simulink model "roll_model_TRUCKSIM_18DOF_REVISED"  (R2023b)
settings: Solver=FixedStepAuto  StartTime=0.0  StopTime=20  FixedStep=0.0005  RelTol=1e-3
StopFcn:
  | save_dataset_18state;
libraries: Solver_SF x1
(part 1 of 5)
settings Model: Creator=duong  LastModifiedBy=ThinkPad
settings SolverCC: AlgebraicLoopSolver=TrustRegion
settings DataIOCC: ReturnWorkspaceOutputs=off
settings SFSimCC: CustomCodeUndefinedFunction=UseInterfaceOnly

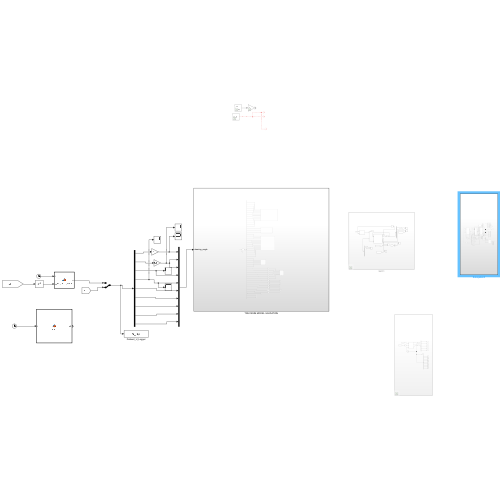
[thumbnail: Simulink's stored preview of the top-level diagram]
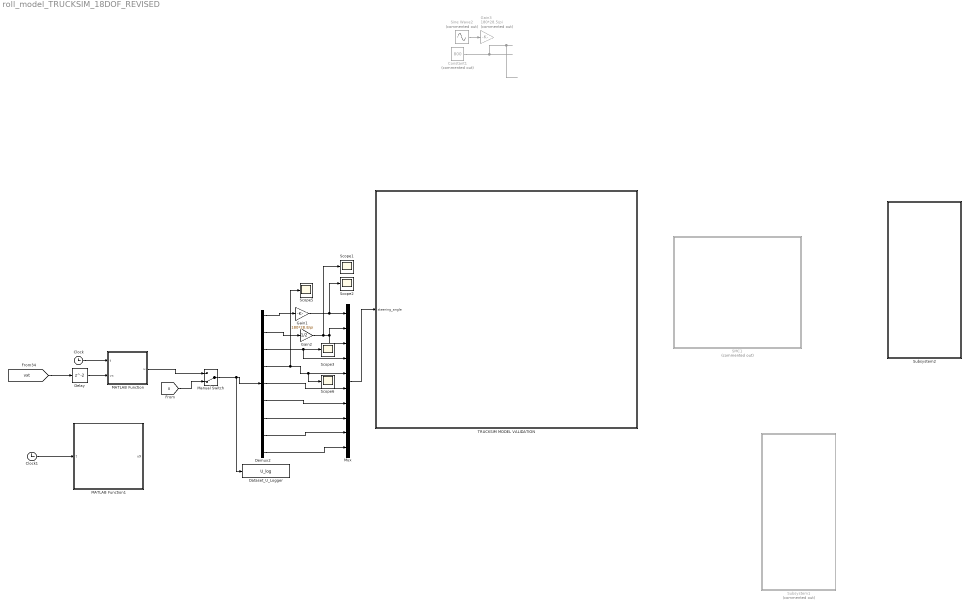
== system roll_model_TRUCKSIM_18DOF_REVISED ==
  Clock : Clock
      settings: Decimation=20
  Clock1 : Clock
      settings: Decimation=20
  Constant1 : Constant  Commented=on  Value=800
  Dataset_U_Logger : ToWorkspace  VariableName=U_log  SampleTime=-1
  Delay : Delay
  Demux2 : Demux  Outputs=9
  Gain1 : Gain  Gain=180*28.8/pi
  Gain2 : Gain  Gain=1/2
  Gain3 : Gain  Commented=on  Gain=180*28.5/pi
  MATLAB Function : MATLAB Function  TreatAsAtomicUnit=on
  MATLAB Function1 : MATLAB Function  TreatAsAtomicUnit=on
  Manual Switch : ManualSwitch  CurrentSetting=0
  Mux : Mux  Inputs=10
  SMC1 : Subsystem  Commented=on
  Scope{1..3,5..6} (5 alike) : Scope
  Sine Wave2 : Sin  Commented=on  Amplitude=0.01  SampleTime=0
  Subsystem1 : Subsystem  Commented=on
  Subsystem2 : Subsystem
  TRUCKSIM MODEL VALIDATION : Subsystem
  wires:
  Mux/1 -> TRUCKSIM MODEL VALIDATION/1(steering_angle)
  Constant1/1 -> ?
  Sine Wave2/1 -> Gain3/1
  Gain2/1 -> Scope1/1, Mux/3, Mux/2
  Demux2/2 -> Gain2/1
  Gain1/1 -> Scope2/1, Mux/1
  Demux2/4 -> Scope5/1, Scope6/1, Mux/5
  Demux2/5 -> Mux/6
  Demux2/6 -> Mux/7
  Demux2/7 -> Mux/8
  Demux2/8 -> Mux/9
  Demux2/9 -> Mux/10
  Clock/1 -> MATLAB Function/1(t)
  [vxt] -> Delay/1
  Delay/1 -> MATLAB Function/2(vx)
  Manual Switch/1 -> Demux2/1, Dataset_U_Logger/1
  [u] -> Manual Switch/2
  Clock1/1 -> MATLAB Function1/1(t)
  Demux2/1 -> Gain1/1
  MATLAB Function/1(u) -> Manual Switch/1
  Demux2/3 -> Mux/4, Scope3/1

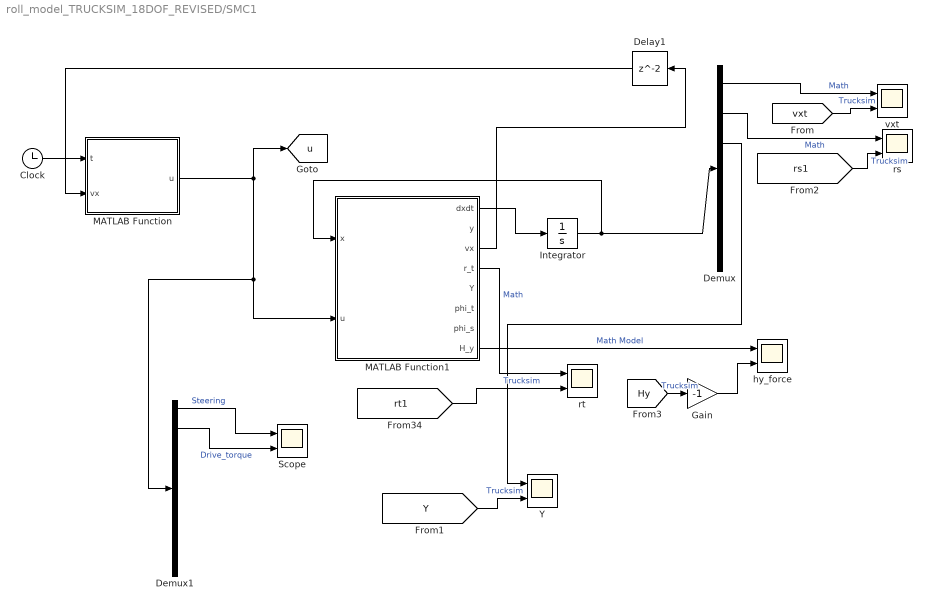
== system roll_model_TRUCKSIM_18DOF_REVISED/SMC1 ==
  Clock : Clock
      settings: Decimation=20
  Delay1 : Delay
  Demux : Demux  Outputs=18
  Demux1 : Demux  Outputs=9
  Gain : Gain  Gain=-1
  Integrator : Integrator  InitialCondition=[12;zeros(7,1);(12/0.51)*ones(6,1);zeros(4,1)]
  MATLAB Function : MATLAB Function  TreatAsAtomicUnit=on
  MATLAB Function1 : MATLAB Function  TreatAsAtomicUnit=on
  Scope : Scope  NumInputPorts=2
  Y : Scope  NumInputPorts=2
  hy_force : Scope  NumInputPorts=2
  rs : Scope  NumInputPorts=2
  rt : Scope  NumInputPorts=2
  vxt : Scope  NumInputPorts=2
  tag scope: u=global
  wires:
  Demux/7 -> Y/1
  MATLAB Function/1(u) -> MATLAB Function1/2(u), Demux1/1, [u]
  Demux1/1 -> Scope/1  "Steering"
  Demux1/2 -> Scope/2  "Drive_torque"
  [rs1] -> rs/2  "Trucksim"
  Demux/4 -> rs/1  "Math"
  [rt1] -> rt/2  "Trucksim"
  [Y] -> Y/2  "Trucksim"
  MATLAB Function1/3(vx) -> Delay1/1
  Delay1/1 -> MATLAB Function/2(vx)
  Demux/1 -> vxt/1  "Math"
  [vxt] -> vxt/2  "Trucksim"
  MATLAB Function1/4(r_t) -> rt/1  "Math"
  Clock/1 -> MATLAB Function/1(t)
  Integrator/1 -> MATLAB Function1/1(x), Demux/1
  MATLAB Function1/1(dxdt) -> Integrator/1
  MATLAB Function1/8(H_y) -> hy_force/1  "Math Model"
  [Hy] -> Gain/1  "Trucksim"
  Gain/1 -> hy_force/2

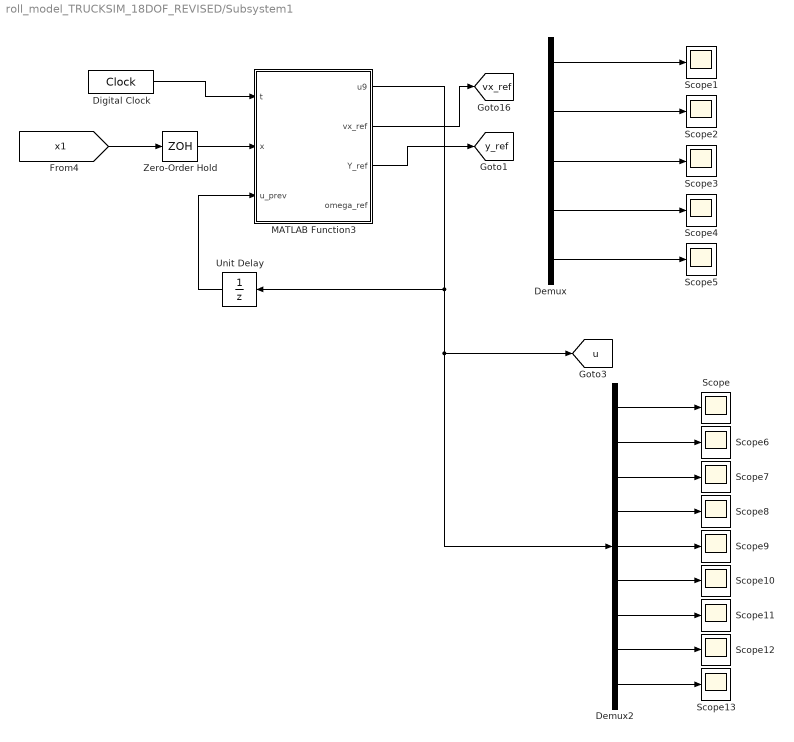
== system roll_model_TRUCKSIM_18DOF_REVISED/Subsystem1 ==
  Demux : Demux  Outputs=5
  Demux2 : Demux  Outputs=9
  Digital Clock : DigitalClock  SampleTime=0.01
  MATLAB Function3 : MATLAB Function  TreatAsAtomicUnit=on
  Scope{,1..13} (14 alike) : Scope
  Unit Delay : UnitDelay  InitialCondition=zeros(9,1)  SampleTime=0.01  HasFrameUpgradeWarning=on
  Zero-Order Hold : ZeroOrderHold  SampleTime=0.01
  tag scope: u=global, vx_ref=global, y_ref=global
  wires:
  Demux2/9 -> Scope13/1
  Demux2/8 -> Scope12/1
  Demux2/7 -> Scope11/1
  Demux2/6 -> Scope10/1
  Demux2/5 -> Scope9/1
  Demux2/4 -> Scope8/1
  Demux2/3 -> Scope7/1
  Demux2/2 -> Scope6/1
  Demux2/1 -> Scope/1
  Demux/5 -> Scope5/1
  Demux/4 -> Scope4/1
  Demux/3 -> Scope3/1
  Demux/2 -> Scope2/1
  Demux/1 -> Scope1/1
  MATLAB Function3/1(u9) -> Unit Delay/1, Demux2/1, [u]
  [x1] -> Zero-Order Hold/1
  Zero-Order Hold/1 -> MATLAB Function3/2(x)
  Unit Delay/1 -> MATLAB Function3/3(u_prev)
  Digital Clock/1 -> MATLAB Function3/1(t)
  MATLAB Function3/2(vx_ref) -> [vx_ref]
  MATLAB Function3/3(Y_ref) -> [y_ref]

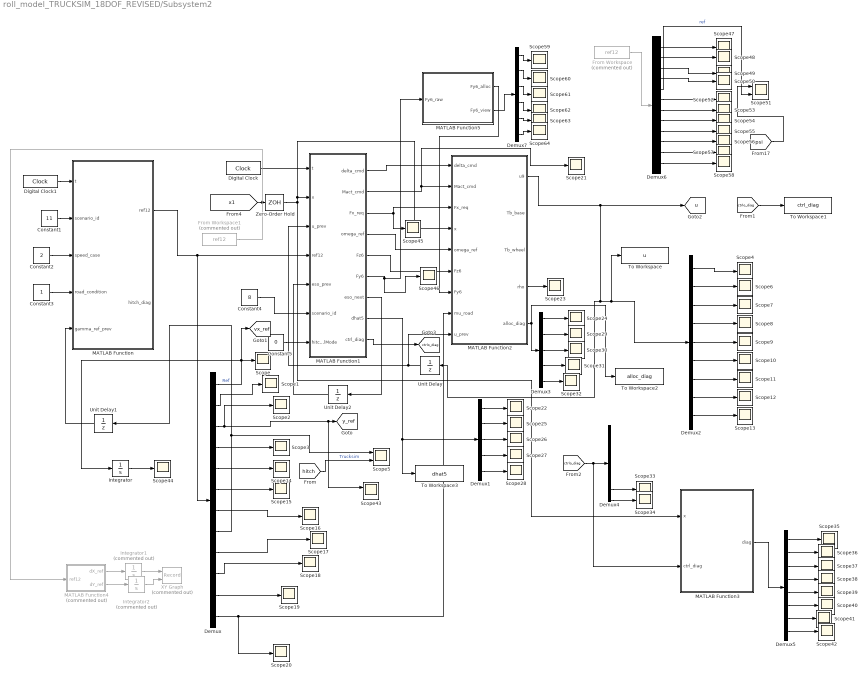
== system roll_model_TRUCKSIM_18DOF_REVISED/Subsystem2 ==
  Constant1 : Constant  Value=11
  Constant2 : Constant  Value=2
  Constant3 : Constant
  Constant4 : Constant  Value=8
  Constant5 : Constant  Value=0
  Demux : Demux  Outputs=12
  Demux1 : Demux  Outputs=5
  Demux2 : Demux  Outputs=9
  Demux3 : Demux  Outputs=5
  Demux4 : Demux  Outputs=8
  Demux5 : Demux  Outputs=8
  Demux6 : Demux  Outputs=12
  Demux7 : Demux  Outputs=6
  Digital Clock : DigitalClock  SampleTime=0.01
  Digital Clock1 : DigitalClock  SampleTime=0.01
  From Workspace : FromWorkspace  Commented=on  VariableName=ref12
  From Workspace1 : FromWorkspace  Commented=on  VariableName=ref12
  Integrator : Integrator
  Integrator1 : Integrator  Commented=on
  Integrator2 : Integrator  Commented=on
  MATLAB Function : MATLAB Function  TreatAsAtomicUnit=on
  MATLAB Function1 : MATLAB Function  TreatAsAtomicUnit=on
  MATLAB Function2 : MATLAB Function  TreatAsAtomicUnit=on
  MATLAB Function3 : MATLAB Function  TreatAsAtomicUnit=on
  MATLAB Function4 : MATLAB Function  Commented=on  TreatAsAtomicUnit=on
  MATLAB Function5 : MATLAB Function  TreatAsAtomicUnit=on
  Scope{,1..4,6..42,44..50,52..64} (62 alike) : Scope
  Scope43 : Scope  NumInputPorts=2
  Scope5 : Scope  NumInputPorts=2
  Scope51 : Scope  NumInputPorts=2
  To Workspace : ToWorkspace  VariableName=u  SaveFormat=Timeseries  SampleTime=-1
  To Workspace1 : ToWorkspace  VariableName=ctrl_diag  SaveFormat=Timeseries  SampleTime=-1
  To Workspace2 : ToWorkspace  VariableName=alloc_diag  SaveFormat=Timeseries  SampleTime=-1
  To Workspace3 : ToWorkspace  VariableName=dhat5  SaveFormat=Timeseries  SampleTime=-1
  Unit Delay : UnitDelay  InitialCondition=zeros(9,1)  SampleTime=0.01  HasFrameUpgradeWarning=on
  Unit Delay1 : UnitDelay  SampleTime=0.01  HasFrameUpgradeWarning=on
  Unit Delay2 : UnitDelay  InitialCondition=zeros(10,1)  SampleTime=0.01  HasFrameUpgradeWarning=on
  XY Graph : Record  Commented=on  FileSettingsInternal="{\"entries\":[{\"content\":{\"excelSettings\":{\"content\":{},\"type\":\"Streamout.ExcelSettings\"}},\"type\":\"Streamout.FileSettingStorage\",\"uuid\":\"\"}],\"packageUris\":[\"http:\\/\\/schema.mathworks.com\\/mf0\\/streamout_blocks\\/R2020a\"],\"version\":\"1.0\"}"  Layout=[1 1]  SignalsInternal="{\"entries\":[{\"content\":{},\"type\":\"RecordBlkView.InputSignals\",\"uuid\":\"\"}],\"packageUris\":[\"http:\\/\\/schema.mathworks.com\\/mf0\\/streamout_blocks\\/R2020a\"],\"version\":\"1.0\"}"  VisualizationBindings="{\"xyplotplugin\":{\"info\":[{\"series\":[],\"subplotID\":1}]}}"  CompatibilityTag=XY
  Zero-Order Hold : ZeroOrderHold  SampleTime=0.01
  tag scope: ctrlo_diag=global, u=global, vx_ref=global, y_ref=global
  wires:
  Digital Clock/1 -> MATLAB Function1/1(t)
  Zero-Order Hold/1 -> MATLAB Function1/2(x), MATLAB Function2/4(x), MATLAB Function3/1(x)
  [x1] -> Zero-Order Hold/1
  Digital Clock1/1 -> MATLAB Function/1(t)
  Constant1/1 -> MATLAB Function/2(scenario_id)
  Constant2/1 -> MATLAB Function/3(speed_case)
  Constant3/1 -> MATLAB Function/4(road_condition)
  MATLAB Function1/1(delta_cmd) -> MATLAB Function2/1(delta_cmd)
  MATLAB Function1/2(Mact_cmd) -> Scope21/1, MATLAB Function2/2(Mact_cmd)
  MATLAB Function1/3(Fx_req) -> Scope45/1, MATLAB Function2/3(Fx_req)
  MATLAB Function1/4(omega_ref) -> MATLAB Function2/5(omega_ref)
  MATLAB Function1/5(Fz6) -> MATLAB Function2/6(Fz6)
  MATLAB Function1/6(Fy6) -> MATLAB Function5/1(Fy6_raw), Scope46/1
  MATLAB Function2/1(u9) -> Unit Delay/1, To Workspace/1, Demux2/1, [u]
  Demux/1 -> [vx_ref], Integrator/1, Scope/1
  Demux/2 -> Scope1/1
  Demux/3 -> Scope2/1, Scope43/1, [y_ref]
  Demux/4 -> Scope3/1
  Unit Delay/1 -> MATLAB Function1/3(u_prev), MATLAB Function2/9(u_prev)
  Demux2/5 -> Scope9/1
  Demux2/2 -> Scope6/1
  Demux2/3 -> Scope7/1
  Demux2/7 -> Scope11/1
  Demux2/1 -> Scope4/1
  Demux2/8 -> Scope12/1
  Demux2/4 -> Scope8/1
  Demux2/6 -> Scope10/1
  Demux2/9 -> Scope13/1
  Demux/8 -> Scope5/1, Unit Delay1/1  "Ref"
  Unit Delay1/1 -> MATLAB Function/5(gamma_ref_prev)
  MATLAB Function1/7(eso_next) -> Unit Delay2/1
  Unit Delay2/1 -> MATLAB Function1/5(eso_prev)
  [hitch] -> Scope5/2  "Trucksim"
  Demux/5 -> Scope14/1
  Demux/6 -> Scope15/1
  Demux/7 -> Scope16/1
  Demux/9 -> Scope17/1
  Demux/10 -> Scope18/1
  Demux/11 -> Scope19/1
  Demux/12 -> MATLAB Function2/8(mu_road), Scope20/1
  MATLAB Function1/8(dhat5) -> To Workspace3/1, Demux1/1
  MATLAB Function2/4(rho) -> Scope23/1
  MATLAB Function2/5(alloc_diag) -> Demux3/1, To Workspace2/1
  Demux1/1 -> Scope22/1
  Demux1/2 -> Scope25/1
  Demux1/3 -> Scope26/1
  Demux1/4 -> Scope27/1
  Demux1/5 -> Scope28/1
  Demux3/1 -> Scope24/1
  Demux3/2 -> Scope29/1
  Demux3/3 -> Scope30/1
  Demux3/4 -> Scope31/1
  Demux3/5 -> Scope32/1
  [ctrlo_diag] -> MATLAB Function3/2(ctrl_diag), Demux4/1
  Demux4/7 -> Scope33/1
  Demux4/8 -> Scope34/1
  MATLAB Function3/1(diag) -> Demux5/1
  Demux5/1 -> Scope35/1
  Demux5/2 -> Scope36/1
  Demux5/3 -> Scope37/1
  Demux5/4 -> Scope38/1
  Demux5/5 -> Scope39/1
  Demux5/6 -> Scope40/1
  Demux5/7 -> Scope41/1
  Demux5/8 -> Scope42/1
  [ctrlo_diag] -> To Workspace1/1
  Integrator/1 -> Scope44/1
  MATLAB Function4/1(dX_ref) -> Integrator1/1
  MATLAB Function4/2(dY_ref) -> Integrator2/1
  Integrator1/1 -> XY Graph/1
  Integrator2/1 -> XY Graph/2
  MATLAB Function1/9(ctrl_diag) -> [ctrlo_diag]
  Constant4/1 -> MATLAB Function1/6(scenario_id)
  From Workspace/1 -> Demux6/1
  Demux6/1 -> Scope47/1
  Demux6/2 -> Scope48/1
  Demux6/3 -> Scope49/1
  Demux6/4 -> Scope50/1
  Demux6/5 -> Scope51/2  "ref"
  Demux6/6 -> Scope52/1
  Demux6/7 -> Scope53/1
  Demux6/8 -> Scope54/1
  Demux6/9 -> Scope55/1
  Demux6/10 -> Scope56/1
  Demux6/11 -> Scope57/1
  Demux6/12 -> Scope58/1
  From Workspace1/1 -> MATLAB Function4/1(ref12)
  [psi] -> Scope51/1
  Constant5/1 -> MATLAB Function1/7(hitchControlMode)
  MATLAB Function5/2(Fy6_view) -> Demux7/1
  Demux7/1 -> Scope59/1
  Demux7/2 -> Scope60/1
  Demux7/3 -> Scope61/1
  Demux7/4 -> Scope62/1
  Demux7/5 -> Scope63/1
  Demux7/6 -> Scope64/1
  MATLAB Function5/1(Fy6_alloc) -> MATLAB Function2/7(Fy6)
  MATLAB Function/1(ref12) -> MATLAB Function1/4(ref12), Demux/1

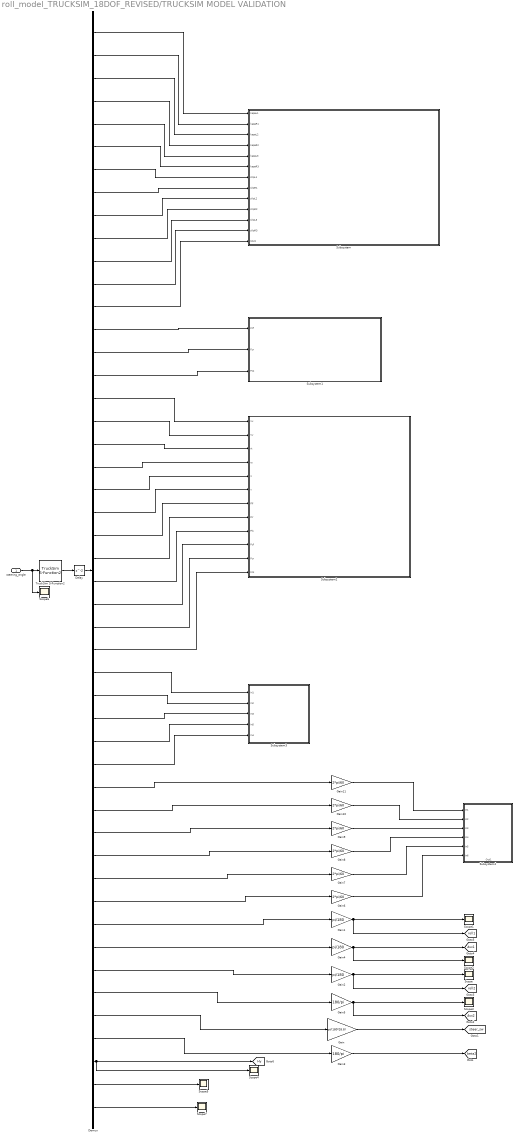
== system roll_model_TRUCKSIM_18DOF_REVISED/TRUCKSIM MODEL VALIDATION ==
  steering_angle : Inport
  Delay : Delay
  Demux : Demux  Outputs=48
  Gain : Gain  Gain=pi/(180*28.8)
  Gain1 : Gain  Gain=pi/180
  Gain{6..11} (6 alike) : Gain  Gain=2*pi/60
  Gain2 : Gain  Gain=pi/180
  Gain3 : Gain  Gain=180/pi
  Gain4 : Gain  Gain=pi/180
  Gain5 : Gain  Gain=180/pi
  Scope{,1..7} (8 alike) : Scope
  Subsystem : Subsystem
  Subsystem1 : Subsystem
  Subsystem2 : Subsystem
  Subsystem3 : Subsystem
  Subsystem4 : Subsystem
      settings: PortSchema="{\"entries\":[{\"content\":{\"sides\":[{\"content\":{\"connectorIds\":[\"In1\",\"In2\",\"In3\",\"In4\",\"In5\",\"In6\"]},\"type\":\"ConnectorPlacement.EquallySpacedRectSide\",\"uuid\":\"070411b8-1eaf-4600-ae67-312ecabb46ce\"},{\"content\":{\"side\":\"RIGHT\"},\"type\":\"ConnectorPlacement.EquallySpacedRectSide\",\"uuid\":\"e64aaffe-29d9-425a-a5f7-83ef24fd6d70\"},{\"content\":{\"side\":\"TOP\"},\"type\":\"ConnectorPlacement.EquallySpacedRectSide\",\"uuid\":\"b5ab375b-6b47-4d88-bc86-a6bac8bdcf5b\"},{\"content\":{\"connectorIds\":[\"Out1\"],\"side\":\"BOTTOM\"},\"type\":\"ConnectorPlacement.EquallySpacedRectSide\",\"uuid\":\"71cf385b-1b44-4da4-ba17-2e03fc073379\"}]},\"type\":\"ConnectorPlacement.EquallySpacedConnector\",\"uuid\":\"3bbbd5e1-cd10-4b5e-b773-54af9b41425b\"}],\"packageUris\":[\"http://schema.mathworks.com/mf0/Connector/R2020b\"],\"version\":\"1.0\"}"
  TruckSim S-Function2 : Solver_SF/TruckSim S-Function2  Priority=1  VehicleCode=s_s  SIMFILE=simfile.sim
      settings: AttributesFormatString=Vehicle Code: %<VehicleCode>  SourceProductName=TruckSim S-Function
  tag scope: Avx1=global, Avx2=global, Hy=global, beta2=global, roll1=global, roll2=global, steer_sw=global
  wires:
  steering_angle/1 -> TruckSim S-Function2/1, Scope6/1
  Demux/19 -> Subsystem2/3(rt)
  Demux/13 -> Subsystem/13(hitch)
  Demux/6 -> Subsystem/6(kapaR3)
  Delay/1 -> Demux/1
  Gain3/1 -> [beta2]
  Demux/35 -> Gain10/1
  Demux/12 -> Subsystem/12(slipR3)
  TruckSim S-Function2/1 -> Delay/1
  Gain11/1 -> Subsystem4/1(In1)
  Demux/40 -> Gain1/1
  Demux/5 -> Subsystem/5(kapaL3)
  Gain10/1 -> Subsystem4/2(In2)
  Demux/18 -> Subsystem2/2(Vy)
  Demux/4 -> Subsystem/4(kapaR2)
  Demux/46 -> Scope4/1, [Hy]
  Demux/29 -> Subsystem3/1(In1)
  Demux/1 -> Subsystem/1(kapaL1)
  Demux/3 -> Subsystem/3(kapaL2)
  Demux/2 -> Subsystem/2(kapaR1)
  Demux/7 -> Subsystem/7(slipL1)
  Gain/1 -> [steer_sw]
  Demux/21 -> Subsystem2/5(X)
  Demux/17 -> Subsystem2/1(Vx)
  Demux/8 -> Subsystem/8(slipR1)
  Demux/9 -> Subsystem/9(slipL2)
  Demux/10 -> Subsystem/10(slipR2)
  Gain7/1 -> Subsystem4/5(In5)
  Demux/39 -> Gain6/1
  Demux/11 -> Subsystem/11(slipL3)
  Demux/44 -> Gain/1
  Demux/36 -> Gain9/1
  Demux/27 -> Subsystem2/11(Fcr)
  Demux/14 -> Subsystem1/1(Fzf)
  Gain4/1 -> [Avx1], Scope2/1
  Gain1/1 -> [roll1], Scope1/1
  Demux/43 -> Gain5/1
  Demux/15 -> Subsystem1/2(Fzr)
  Gain9/1 -> Subsystem4/3(In3)
  Demux/32 -> Subsystem3/4(In5)
  Demux/16 -> Subsystem1/3(Fzs)
  Demux/42 -> Gain2/1
  Demux/26 -> Subsystem2/10(Fcf)
  Demux/20 -> Subsystem2/4(rs)
  Gain6/1 -> Subsystem4/6(In6)
  Demux/38 -> Gain7/1
  Demux/28 -> Subsystem2/12(Fcs)
  Demux/22 -> Subsystem2/6(Y)
  Demux/30 -> Subsystem3/2(In2)
  Demux/23 -> Subsystem2/7(Flf)
  Demux/41 -> Gain4/1
  Demux/24 -> Subsystem2/8(Flr)
  Gain8/1 -> Subsystem4/4(In4)
  Demux/45 -> Gain3/1
  Demux/25 -> Subsystem2/9(Fls)
  Demux/37 -> Gain8/1
  Demux/33 -> Subsystem3/5(In4)
  Demux/31 -> Subsystem3/3(In3)
  Demux/34 -> Gain11/1
  Gain5/1 -> Scope3/1, [Avx2]
  Gain2/1 -> Scope/1, [roll2]
  Demux/47 -> Scope5/1
  Demux/48 -> Scope7/1

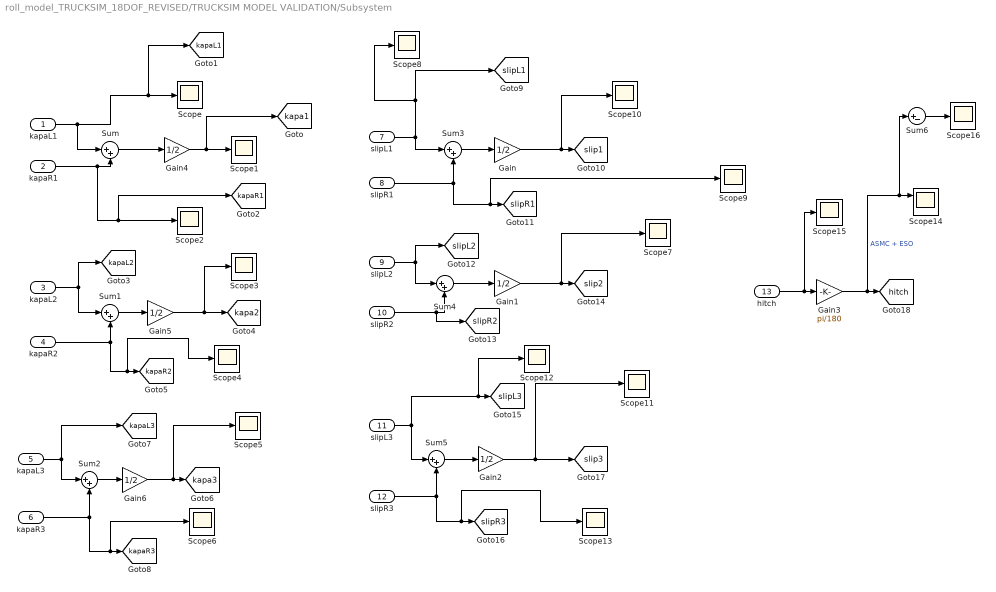
== system roll_model_TRUCKSIM_18DOF_REVISED/TRUCKSIM MODEL VALIDATION/Subsystem ==
  kapaL1 : Inport
  kapaR1 : Inport  Port=2
  kapaL2 : Inport  Port=3
  kapaR2 : Inport  Port=4
  kapaL3 : Inport  Port=5
  kapaR3 : Inport  Port=6
  slipL1 : Inport  Port=7
  slipR1 : Inport  Port=8
  slipL2 : Inport  Port=9
  slipR2 : Inport  Port=10
  slipL3 : Inport  Port=11
  slipR3 : Inport  Port=12
  hitch : Inport  Port=13
  Gain{,1..2,4..6} (6 alike) : Gain  Gain=1/2
  Gain3 : Gain  Gain=pi/180
  Scope{,1..13,15..16} (16 alike) : Scope
  Scope14 : Scope  NumInputPorts=2
  Sum{,1..5} (6 alike) : Sum  Inputs=|++
  Sum6 : Sum  Inputs=|+-
  tag scope: hitch=global, kapa1=global, kapa2=global, kapa3=global, kapaL1=global, kapaL2=global, kapaL3=global, kapaR1=global, kapaR2=global, kapaR3=global, slip1=global, slip2=global, slip3=global, slipL1=global, slipL2=global, slipL3=global, slipR1=global, slipR2=global, slipR3=global
  wires:
  kapaL1/1 -> Scope/1, [kapaL1], Sum/1
  kapaR1/1 -> [kapaR1], Scope2/1, Sum/2
  Sum/1 -> Gain4/1
  kapaL2/1 -> [kapaL2], Sum1/1
  kapaR2/1 -> Scope4/1, [kapaR2], Sum1/2
  Sum1/1 -> Gain5/1
  kapaL3/1 -> [kapaL3], Sum2/1
  kapaR3/1 -> Scope6/1, [kapaR3], Sum2/2
  Sum2/1 -> Gain6/1
  slipL1/1 -> Scope8/1, [slipL1], Sum3/1
  slipR1/1 -> Scope9/1, [slipR1], Sum3/2
  Sum3/1 -> Gain/1
  Gain/1 -> Scope10/1, [slip1]
  slipL2/1 -> [slipL2], Sum4/1
  slipR2/1 -> [slipR2], Sum4/2
  Sum4/1 -> Gain1/1
  Gain1/1 -> Scope7/1, [slip2]
  slipL3/1 -> Scope12/1, [slipL3], Sum5/1
  slipR3/1 -> Scope13/1, [slipR3], Sum5/2
  Sum5/1 -> Gain2/1
  Gain2/1 -> Scope11/1, [slip3]
  hitch/1 -> Scope15/1, Gain3/1
  Gain3/1 -> Sum6/1, Scope14/1, [hitch]  "ASMC + ESO"
  Gain4/1 -> [kapa1], Scope1/1
  Gain5/1 -> [kapa2], Scope3/1
  Gain6/1 -> Scope5/1, [kapa3]
  Sum6/1 -> Scope16/1

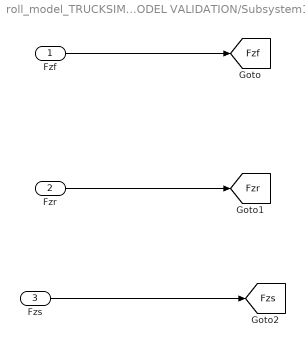
== system roll_model_TRUCKSIM_18DOF_REVISED/TRUCKSIM MODEL VALIDATION/Subsystem1 ==
  Fzf : Inport
  Fzr : Inport  Port=2
  Fzs : Inport  Port=3
  tag scope: Fzf=global, Fzr=global, Fzs=global
  wires:
  Fzf/1 -> [Fzf]
  Fzr/1 -> [Fzr]
  Fzs/1 -> [Fzs]

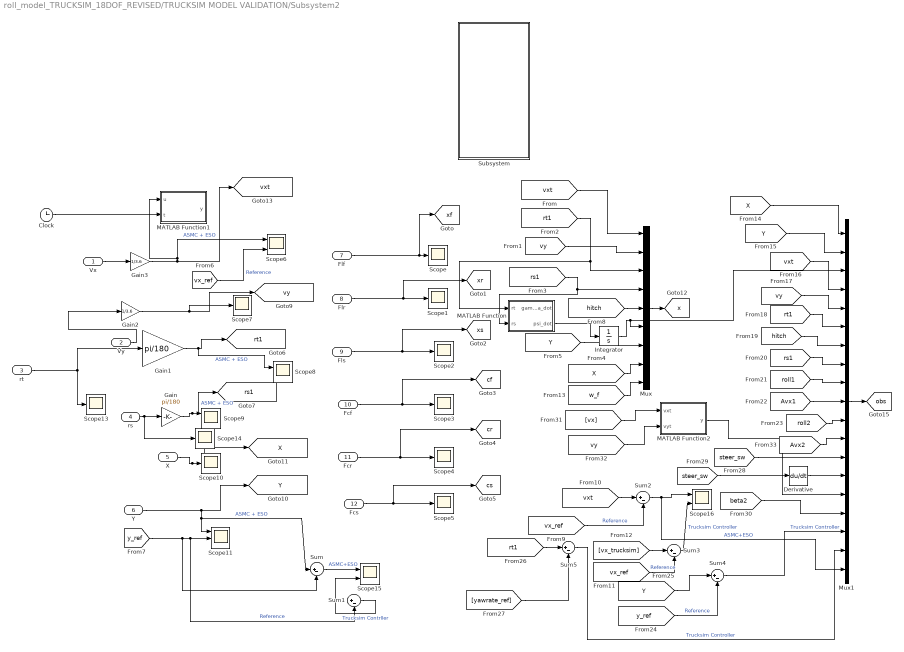
== system roll_model_TRUCKSIM_18DOF_REVISED/TRUCKSIM MODEL VALIDATION/Subsystem2 ==
  Vx : Inport
  Vy : Inport  Port=2
  rt : Inport  Port=3
  rs : Inport  Port=4
  X : Inport  Port=5
  Y : Inport  Port=6
  Flf : Inport  Port=7
  Flr : Inport  Port=8
  Fls : Inport  Port=9
  Fcf : Inport  Port=10
  Fcr : Inport  Port=11
  Fcs : Inport  Port=12
  Clock : Clock
      settings: Decimation=15
  Derivative : Derivative
  Gain : Gain  Gain=pi/180
  Gain1 : Gain  Gain=pi/180
  Gain2 : Gain  Gain=1/3.6
  Gain3 : Gain  Gain=1/3.6
  Integrator : Integrator
  MATLAB Function : MATLAB Function  TreatAsAtomicUnit=on
  MATLAB Function1 : MATLAB Function  TreatAsAtomicUnit=on
  MATLAB Function2 : MATLAB Function  TreatAsAtomicUnit=on
  Mux : Mux  Inputs=9
  Mux1 : Mux  Inputs=19
  Scope{,1..5,7,10,13..14} (10 alike) : Scope
  Scope11 : Scope  NumInputPorts=3
  Scope{6,8..9,15..16} (5 alike) : Scope  NumInputPorts=2
  Subsystem : Subsystem
  Sum{,1..5} (6 alike) : Sum  Inputs=|+-
  tag scope: X=global, Y=global, cf=global, cr=global, cs=global, obs=global, rs1=global, rt1=global, vxt=global, vy=global, x=global, xf=global, xr=global, xs=global
  wires:
  Fcf/1 -> [cf], Scope3/1
  Fcr/1 -> [cr], Scope4/1
  Fcs/1 -> [cs], Scope5/1
  Vx/1 -> Gain3/1
  Vy/1 -> Gain2/1
  rt/1 -> Scope13/1, Gain1/1
  rs/1 -> Scope14/1, Gain/1
  X/1 -> [X], Scope10/1
  Y/1 -> [Y], Scope11/1, Sum/1  "ASMC + ESO"
  Gain/1 -> [rs1], Scope9/1  "ASMC + ESO"
  Gain1/1 -> Scope8/1, [rt1]  "ASMC + ESO"
  Flr/1 -> [xr], Scope1/1
  Flf/1 -> [xf], Scope/1
  Fls/1 -> [xs], Scope2/1
  Gain2/1 -> [vy], Scope7/1
  Gain3/1 -> Scope6/1, MATLAB Function1/1(u), [vxt]  "ASMC + ESO"
  Clock/1 -> MATLAB Function1/2(t)
  [vxt] -> Mux/1
  [vy] -> Mux/2
  [rt1] -> Mux/3, MATLAB Function/1(rt)
  [rs1] -> Mux/4, MATLAB Function/2(rs)
  [X] -> Mux/8
  [Y] -> Mux/7
  Mux/1 -> [x]
  [y_ref] -> Sum/2, Sum1/2, Scope11/2  "Reference"
  [hitch] -> Mux/5
  Integrator/1 -> Mux1/3, Mux/6
  MATLAB Function/2(psi_dot) -> Integrator/1
  Sum/1 -> Scope15/1  "ASMC+ESO"
  Sum1/1 -> Scope15/2  "Trucksim Contrller"
  [vx_ref] -> Sum2/2  "Reference"
  [vxt] -> Sum2/1
  [vx_ref] -> Sum3/2  "Reference"
  [vx_trucksim] -> Sum3/1
  Sum2/1 -> Mux1/19, Scope16/1  "ASMC+ESO"
  Sum3/1 -> Scope16/2  "Trucksim Controller"
  [w_f] -> Mux/9
  [X] -> Mux1/1
  [Y] -> Mux1/2
  [vxt] -> Mux1/4
  [vy] -> Mux1/5
  [rt1] -> Mux1/6
  Mux1/1 -> [obs]
  [Y] -> Sum4/1
  [y_ref] -> Sum4/2  "Reference"
  Sum4/1 -> Mux1/17  "Trucksim Controller"
  [rt1] -> Sum5/1
  [yawrate_ref] -> Sum5/2
  Sum5/1 -> Mux1/18  "Trucksim Controller"
  [hitch] -> Mux1/7
  [rs1] -> Mux1/8
  [roll1] -> Mux1/9
  [Avx1] -> Mux1/10
  [roll2] -> Mux1/11
  [steer_sw] -> Derivative/1
  [beta2] -> Mux1/16
  [vx] -> MATLAB Function2/1(vxt)
  [vy] -> MATLAB Function2/2(vyt)
  MATLAB Function2/1(y) -> Mux1/15
  Derivative/1 -> Mux1/14
  [steer_sw] -> Mux1/13
  [Avx2] -> Mux1/12
  [vx_ref] -> Scope6/2  "Reference"

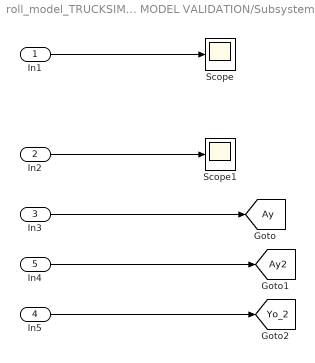
== system roll_model_TRUCKSIM_18DOF_REVISED/TRUCKSIM MODEL VALIDATION/Subsystem3 ==
  In1 : Inport
  In2 : Inport  Port=2
  In3 : Inport  Port=3
  In5 : Inport  Port=4
  In4 : Inport  Port=5
  Scope : Scope
  Scope1 : Scope
  tag scope: Ay2=global, Ay=global, Yo_2=global
  wires:
  In2/1 -> Scope1/1
  In1/1 -> Scope/1
  In3/1 -> [Ay]
  In4/1 -> [Ay2]
  In5/1 -> [Yo_2]

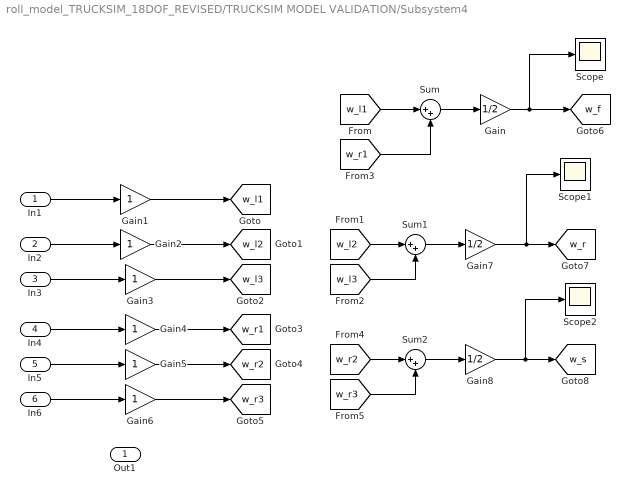
== system roll_model_TRUCKSIM_18DOF_REVISED/TRUCKSIM MODEL VALIDATION/Subsystem4 ==
  In1 : Inport
  In2 : Inport  Port=2
  In3 : Inport  Port=3
  In4 : Inport  Port=4
  In5 : Inport  Port=5
  In6 : Inport  Port=6
  Gain : Gain  Gain=1/2
  Gain{1..6} (6 alike) : Gain
  Gain7 : Gain  Gain=1/2
  Gain8 : Gain  Gain=1/2
  Scope : Scope
  Scope1 : Scope
  Scope2 : Scope
  Sum : Sum  Inputs=|++
  Sum1 : Sum  Inputs=|++
  Sum2 : Sum  Inputs=|++
  Out1 : Outport
  tag scope: w_f=global, w_l1=global, w_l2=global, w_l3=global, w_r1=global, w_r2=global, w_r3=global, w_r=global, w_s=global
  wires:
  [w_l1] -> Sum/1
  [w_r1] -> Sum/2
  Sum/1 -> Gain/1
  In1/1 -> Gain1/1
  Gain1/1 -> [w_l1]
  In2/1 -> Gain2/1
  Gain2/1 -> [w_l2]
  In3/1 -> Gain3/1
  Gain3/1 -> [w_l3]
  In4/1 -> Gain4/1
  Gain4/1 -> [w_r1]
  In5/1 -> Gain5/1
  Gain5/1 -> [w_r2]
  In6/1 -> Gain6/1
  Gain6/1 -> [w_r3]
  Gain/1 -> Scope/1, [w_f]
  Gain7/1 -> Scope1/1, [w_r]
  [w_l2] -> Sum1/1
  Sum1/1 -> Gain7/1
  [w_l3] -> Sum1/2
  Gain8/1 -> Scope2/1, [w_s]
  [w_r2] -> Sum2/1
  Sum2/1 -> Gain8/1
  [w_r3] -> Sum2/2

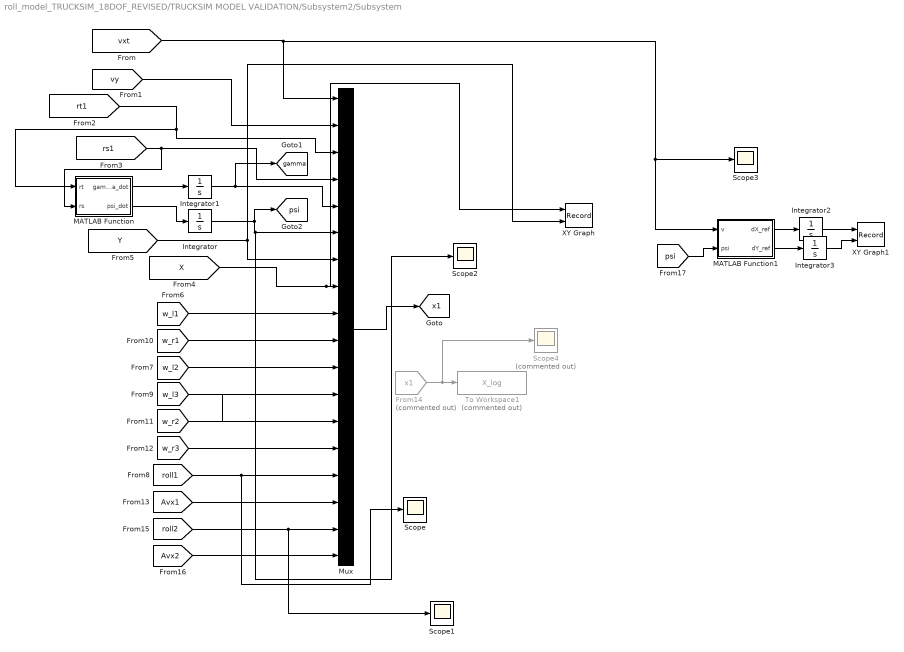
== system roll_model_TRUCKSIM_18DOF_REVISED/TRUCKSIM MODEL VALIDATION/Subsystem2/Subsystem ==
  From14 : From  Commented=on  GotoTag=x1  TagVisibility=global
  Integrator{,1..3} (4 alike) : Integrator
  MATLAB Function : MATLAB Function  TreatAsAtomicUnit=on
  MATLAB Function1 : MATLAB Function  TreatAsAtomicUnit=on
  Mux : Mux  Inputs=18
  Scope{,1..3} (4 alike) : Scope
  Scope4 : Scope  Commented=on
  To Workspace1 : ToWorkspace  Commented=on  VariableName=X_log  SampleTime=-1
  XY Graph : Record  FileSettingsInternal="{\"entries\":[{\"content\":{\"excelSettings\":{\"content\":{},\"type\":\"Streamout.ExcelSettings\"}},\"type\":\"Streamout.FileSettingStorage\",\"uuid\":\"\"}],\"packageUris\":[\"http:\\/\\/schema.mathworks.com\\/mf0\\/streamout_blocks\\/R2020a\"],\"version\":\"1.0\"}"  Layout=[1 1]  SignalsInternal="{\"entries\":[{\"content\":{\"signals\":[{\"content\":{\"blockPath\":[],\"dimensions\":[1],\"domain\":\"\",\"lineColor\":\"#a2142f\",\"plots\":[1],\"port\":1,\"sid\":[\"\"],\"signalID\":8528,\"signalName\":\"From4\"},\"type\":\"RecordBlkView.Signal\",\"uuid\":\"\"},{\"content\":{\"blockPath\":[],\"dimensions\":[1],\"domain\":\"\",\"lineColor\":\"#139fff\",\"plots\":[1],\"port\":2,\"sid\":[\"\"],\"signalID\":8532,\"signalName\":\"From5\"},\"type\":\"RecordBlkView.Signal\",\"uuid\":\"\"}]},\"type\":\"RecordBlkView.InputSignals\",\"uuid\":\"\"}],\"packageUris\":[\"http:\\/\\/schema.mathworks.com\\/mf0\\/streamout_blocks\\/R2020a\"],\"version\":\"1.0\"}"  VisualizationBindings="{\"xyplotplugin\":{\"info\":[{\"series\":[{\"bindingParametersList\":[{\"parameter\":\"X-Axis\",\"signalID\":8528,\"signalName\":\"From4\"},{\"parameter\":\"Y-Axis\",\"signalID\":8532,\"signalName\":\"From5\"}],\"seriesID\":4705}],\"subplotID\":1}]}}"  CompatibilityTag=XY
  XY Graph1 : Record  FileSettingsInternal="{\"entries\":[{\"content\":{\"excelSettings\":{\"content\":{},\"type\":\"Streamout.ExcelSettings\"}},\"type\":\"Streamout.FileSettingStorage\",\"uuid\":\"\"}],\"packageUris\":[\"http:\\/\\/schema.mathworks.com\\/mf0\\/streamout_blocks\\/R2020a\"],\"version\":\"1.0\"}"  Layout=[1 1]  SignalsInternal="{\"entries\":[{\"content\":{\"signals\":[{\"content\":{\"blockPath\":[],\"dimensions\":[1],\"domain\":\"\",\"lineColor\":\"#a2142f\",\"plots\":[1],\"port\":1,\"sid\":[\"\"],\"signalID\":8536,\"signalName\":\"Integrator2\"},\"type\":\"RecordBlkView.Signal\",\"uuid\":\"\"},{\"content\":{\"blockPath\":[],\"dimensions\":[1],\"domain\":\"\",\"lineColor\":\"#139fff\",\"plots\":[1],\"port\":2,\"sid\":[\"\"],\"signalID\":8540,\"signalName\":\"Integrator3\"},\"type\":\"RecordBlkView.Signal\",\"uuid\":\"\"}]},\"type\":\"RecordBlkView.InputSignals\",\"uuid\":\"\"}],\"packageUris\":[\"http:\\/\\/schema.mathworks.com\\/mf0\\/streamout_blocks\\/R2020a\"],\"version\":\"1.0\"}"  VisualizationBindings="{\"xyplotplugin\":{\"info\":[{\"series\":[{\"bindingParametersList\":[{\"parameter\":\"X-Axis\",\"signalID\":8536,\"signalName\":\"Integrator2\"},{\"parameter\":\"Y-Axis\",\"signalID\":8540,\"signalName\":\"Integrator3\"}],\"seriesID\":29226}],\"subplotID\":1}]}}"  CompatibilityTag=XY
  tag scope: gamma=global, psi=global, x1=global
  wires:
  MATLAB Function/2(psi_dot) -> Integrator/1
  [vy] -> Mux/2
  [X] -> XY Graph/1, Mux/8
  Integrator/1 -> [psi], Scope2/1, Mux/6
  [Y] -> XY Graph/2, Mux/7
  [rs1] -> MATLAB Function/2(rs), Mux/4
  [vxt] -> MATLAB Function1/1(v), Scope3/1, Mux/1
  [rt1] -> MATLAB Function/1(rt), Mux/3
  MATLAB Function/1(gamma_dot) -> Integrator1/1
  Integrator1/1 -> [gamma], Mux/5
  [w_l1] -> Mux/9
  [w_r1] -> Mux/10
  [w_l2] -> Mux/11
  [w_r3] -> Mux/14
  [roll1] -> Scope/1, Mux/15
  [Avx1] -> Mux/16
  Mux/1 -> [x1]
  From14/1 -> Scope4/1, To Workspace1/1
  [w_r2] -> Mux/12
  [w_l3] -> Mux/13
  [roll2] -> Scope1/1, Mux/17
  [Avx2] -> Mux/18
  [psi] -> MATLAB Function1/2(psi)
  MATLAB Function1/1(dX_ref) -> Integrator2/1
  Integrator2/1 -> XY Graph1/1
  MATLAB Function1/2(dY_ref) -> Integrator3/1
  Integrator3/1 -> XY Graph1/2

== matlab function roll_model_TRUCKSIM_18DOF_REVISED/Subsystem2/MATLAB Function3 ==
  data: x input; diag output; ctrl_diag input
function diag = fcn(x,ctrl_diag)
%#codegen

phi_t  = x(15);
dphi_t = x(16);

phi_s  = x(17);
dphi_s = x(18);

sPhiT = dphi_t + 3.0*phi_t;
sPhiS = dphi_s + 2.0*phi_s;

sRoll_calc = sPhiT + 0.30*sPhiS;

diag = zeros(8,1);

diag(1) = phi_t;
diag(2) = dphi_t;
diag(3) = phi_s;
diag(4) = dphi_s;

diag(5) = sPhiT;
diag(6) = sPhiS;
diag(7) = sRoll_calc;
diag(8) = sRoll_calc - ctrl_diag(7);
end

== matlab function roll_model_TRUCKSIM_18DOF_REVISED/Subsystem1/MATLAB Function3 ==
  data: t input; u9 output; x input; u_prev input; vx_ref output; Y_ref output; omega_ref output
function [u9,vx_ref,Y_ref,omega_ref] = fcn(t,x,u_prev)
%#codegen
% =========================================================================
% MODEL-ASSISTED SMC FOR FULL 18-STATE TRACTOR-SEMITRAILER
%
% FULL MODEL:
%   vehicle_18dof_full_roll(x,u)
%
% STATES:
% x(1)  = vx
% x(2)  = vy
% x(3)  = rt
% x(4)  = rs
% x(5)  = gamma
% x(6)  = psi
% x(7)  = Y
% x(8)  = X
%
% x(9)  = omega_fL
% x(10) = omega_fR
% x(11) = omega_rL
% x(12) = omega_rR
% x(13) = omega_sL
% x(14) = omega_sR
%
% x(15:18) = roll states
%
% PHYSICAL INPUT:
% u9(1) = delta
% u9(2) = Tdrive
% u9(3) = Mact
% u9(4) = Tb_fL
% u9(5) = Tb_fR
% u9(6) = Tb_rL
% u9(7) = Tb_rR
% u9(8) = Tb_sL
% u9(9) = Tb_sR
% =========================================================================


%% ========================================================================
% FIXED OUTPUT DIMENSIONS
% ========================================================================

u9 = zeros(9,1);

omega_ref = zeros(6,1);


%% ========================================================================
% CONTROLLER SAMPLE TIME
% ========================================================================

Ts = 0.01;


%% ========================================================================
% STATES
% ========================================================================

vx = x(1);

vy = x(2);

rt = x(3);

rs = x(4);

gamma = x(5);

psi = x(6);

Y = x(7);


omega_fL = x(9);
omega_fR = x(10);

omega_rL = x(11);
omega_rR = x(12);

omega_sL = x(13);
omega_sR = x(14);

% Roll states
phi_t  = x(15);
dphi_t = x(16);
phi_s  = x(17);
dphi_s = x(18);


%% ========================================================================
% REFERENCE GENERATOR
% ========================================================================

[vx_ref,ax_ref,Y_ref,dY_ref,psi_ref,rt_ref] = ...
    reference_local(t);


%% Reference one step ahead

[~,~,~,~,~,rt_ref_next] = ...
    reference_local(t+Ts);


dr_ref = ...
    (rt_ref_next-rt_ref)/Ts;


%% ========================================================================
% FULL 18-STATE MODEL
%
% This is the important difference from the previous simple SMC.
%
% The controller now explicitly uses the nonlinear plant model.
% ========================================================================

[xdot_model,y_model] = ...
    vehicle_18dof_full_roll(x,u_prev);


%% Model-predicted accelerations

ax_model = ...
    xdot_model(1);


dr_model = ...
    xdot_model(3);


Ydot_model = ...
    xdot_model(7);

% Model-predicted roll accelerations
ddphi_t_model = xdot_model(16);
ddphi_s_model = xdot_model(18);

% Model-predicted load-transfer ratios
LTR_f_model = y_model(6);
LTR_r_model = y_model(7);
LTR_s_model = y_model(47); %#ok<NASGU>

if abs(LTR_f_model) >= abs(LTR_r_model)
    LTR_t_model = LTR_f_model;
else
    LTR_t_model = LTR_r_model;
end


%% ========================================================================
% VEHICLE PARAMETERS
% ========================================================================

m_t = 5760.0;

m_s = 6640.0;

m = ...
    m_t+m_s;


%% Geometry

Lf = 1.305130208;

Lr = 2.194869792;

L = ...
    Lf+Lr;


Tf = 2.030;

Tr = 1.863;

Ts_track = 1.863;


%% Wheel radii

Rf = 0.51;

Rr = 0.51;

Rs = 0.51;


%% ========================================================================
% 1. MODEL-ASSISTED LONGITUDINAL SMC
% ========================================================================

ev = ...
    vx-vx_ref;


%% Desired longitudinal acceleration

kv = ...
    29.2;


Kv = ...
    2.75;


phi_v = ...
    0.6;


ax_des = ...
      ax_ref ...
    - kv*ev ...
    - Kv*satfun(ev/phi_v);


%% ------------------------------------------------------------------------
% Convert previous physical actuators to approximate total Fx
% -------------------------------------------------------------------------

Fx_prev = ...
    u_prev(2)/Rf;


Fx_prev = ...
    Fx_prev ...
    - u_prev(4)/Rf ...
    - u_prev(5)/Rf ...
    - u_prev(6)/Rr ...
    - u_prev(7)/Rr ...
    - u_prev(8)/Rs ...
    - u_prev(9)/Rs;


%% ------------------------------------------------------------------------
% Model-assisted correction
%
% Delta Fx = m * (desired acceleration - model acceleration)
% -------------------------------------------------------------------------

dFx = ...
    m*(ax_des-ax_model);


Fx_target = ...
    Fx_prev+dFx;


%% Force limits

if Fx_target > 15000.0

    Fx_target = 15000.0;

elseif Fx_target < -15000.0

    Fx_target = -15000.0;

end


%% ========================================================================
% 2. MODEL-ASSISTED LATERAL SMC
% ========================================================================

eY = ...
    Y-Y_ref;


eYdot = ...
    Ydot_model-dY_ref;


epsi = ...
    wrap_pi(psi-psi_ref);


er = ...
    rt-rt_ref;


%% Sliding surface

lambda_Y = ...
    0.90;


lambda_Ydot = ...
    0.82;


lambda_psi = ...
    1.00;


s_lat = ...
      er ...
    + lambda_psi*epsi ...
    + lambda_Y*eY ...
    + lambda_Ydot*eYdot;


%% ========================================================================
% DESIRED YAW ACCELERATION
% ========================================================================

Kr = ...
    2.5;


Kpsi = ...
    1.2;


KY = ...
    0.4;


KYdot = ...
    0.35;


Ksw = ...
    0.7;


phi_lat = ...
    0.2;


dr_des = ...
      dr_ref ...
    - Kr*er ...
    - Kpsi*epsi ...
    - KY*eY ...
    - KYdot*eYdot ...
    - Ksw*satfun(s_lat/phi_lat);


%% ========================================================================
% STEERING SENSITIVITY FROM FULL NONLINEAR MODEL
%
% Numerically estimate:
%
%       d(dr_t)/d(delta)
%
% using vehicle_18dof_full_roll itself.
% ========================================================================

delta_previous = ...
    u_prev(1);


delta_probe = ...
    0.20*pi/180.0;


u_probe = ...
    u_prev;


delta_probe_value = ...
    delta_previous+delta_probe;


delta_max = ...
    5.0*pi/180.0;


if delta_probe_value > delta_max

    delta_probe_value = delta_max;

end


u_probe(1) = ...
    delta_probe_value;


xdot_probe = ...
    vehicle_18dof_full_roll(x,u_probe);


dr_probe = ...
    xdot_probe(3);


d_delta = ...
    delta_probe_value-delta_previous;


if abs(d_delta) > 1.0e-8

    Bdelta = ...
        (dr_probe-dr_model)/d_delta;

else

    Bdelta = ...
        0.0;

end


%% ========================================================================
% MODEL-INVERSE STEERING
% ========================================================================

if abs(Bdelta) > 0.20

    delta_model = ...
        delta_previous ...
        +(dr_des-dr_model)/Bdelta;

else

    delta_model = ...
        delta_previous;

end


%% Limit model inversion

if delta_model > delta_max

    delta_model = delta_max;

elseif delta_model < -delta_max

    delta_model = -delta_max;

end


%% ========================================================================
% DIRECT SMC STEERING
%
% Backup / stabilizing component
% ========================================================================

vx_safe = ...
    max(abs(vx),3.0);


delta_ff = ...
    atan(L*rt_ref/vx_safe);


Kdelta = ...
   2*pi/180.0;


delta_direct = ...
      delta_ff ...
    - 0.18*epsi ...
    - 0.010*eY ...
    - 0.015*eYdot ...
    - Kdelta*satfun(s_lat/phi_lat);


%% Limit

if delta_direct > delta_max

    delta_direct = delta_max;

elseif delta_direct < -delta_max

    delta_direct = -delta_max;

end


%% ========================================================================
% BLEND MODEL-INVERSE + DIRECT SMC
% ========================================================================

if abs(Bdelta) > 0.20

    alpha_model = ...
        0.15;

else

    alpha_model = ...
        0.0;

end


delta_target = ...
      alpha_model*delta_model ...
    + (1.0-alpha_model)*delta_direct;


%% Final steering saturation

if delta_target > delta_max

    delta_target = delta_max;

elseif delta_target < -delta_max

    delta_target = -delta_max;

end


%% ========================================================================
% STEERING RATE LIMIT
% ========================================================================

delta_rate_max = ...
    12.0*pi/180.0;


delta_step_max = ...
    delta_rate_max*Ts;


delta_cmd = ...
    rate_limit( ...
        delta_target, ...
        delta_previous, ...
        delta_step_max );


%% ========================================================================
% 3. MODEL-ASSISTED ACTIVE ROLL SMC
% ========================================================================

phi_t_ref = 0.0;
phi_s_ref = 0.0;

ephi_t = phi_t-phi_t_ref;
ephi_s = phi_s-phi_s_ref;

lambda_phi_t = 3.0;
lambda_phi_s = 2.0;

s_phi_t = dphi_t + lambda_phi_t*ephi_t;
s_phi_s = dphi_s + lambda_phi_s*ephi_s;

w_phi_s = 0.30;

s_roll = s_phi_t + w_phi_s*s_phi_s;

% Desired roll accelerations
k_phi_t   = 1.8;
eta_phi_t = 0.70;
phi_bl_t  = 0.040;

ddphi_t_des = ...
      -lambda_phi_t*dphi_t ...
      -k_phi_t*s_phi_t ...
      -eta_phi_t*satfun(s_phi_t/phi_bl_t);

k_phi_s   = 1.0;
eta_phi_s = 0.35;
phi_bl_s  = 0.050;

ddphi_s_des = ...
      -lambda_phi_s*dphi_s ...
      -k_phi_s*s_phi_s ...
      -eta_phi_s*satfun(s_phi_s/phi_bl_s);

% Mact limits / probe
Mact_max   = 15000.0;
Mact_probe = 500.0;

u_roll_probe = u_prev;

if u_prev(3) > (Mact_max-Mact_probe)
    u_roll_probe(3) = u_prev(3)-Mact_probe;
else
    u_roll_probe(3) = u_prev(3)+Mact_probe;
end

u_roll_probe(3) = clamp(u_roll_probe(3),-Mact_max,Mact_max);

dMact_probe = u_roll_probe(3)-u_prev(3);

if abs(dMact_probe) > 1.0e-9

    [xdot_roll_probe,y_roll_probe] = ...
        vehicle_18dof_full_roll(x,u_roll_probe);

    B_phi_t = ...
        (xdot_roll_probe(16)-ddphi_t_model)/dMact_probe;

    B_phi_s = ...
        (xdot_roll_probe(18)-ddphi_s_model)/dMact_probe;

    if abs(y_roll_probe(6)) >= abs(y_roll_probe(7))
        LTR_t_probe = y_roll_probe(6);
    else
        LTR_t_probe = y_roll_probe(7);
    end

    B_LTR = ...
        (LTR_t_probe-LTR_t_model)/dMact_probe;

else

    B_phi_t = 0.0;
    B_phi_s = 0.0;
    B_LTR   = 0.0;

end

B_roll = B_phi_t + w_phi_s*B_phi_s;

% Model-inverse component
roll_acc_error = ...
      (ddphi_t_des-ddphi_t_model) ...
    + w_phi_s*(ddphi_s_des-ddphi_s_model);

if abs(B_roll) > 1.0e-8
    Mact_model = ...
        u_prev(3) + roll_acc_error/B_roll;
else
    Mact_model = ...
        u_prev(3);
end

Mact_model = clamp(Mact_model,-Mact_max,Mact_max);

% Robust SMC component
if B_roll < 0.0
    sign_Broll = -1.0;
else
    sign_Broll = 1.0;
end

K_Mact_sw  = 4500.0;
K_Mact_lin = 7000.0;
phi_roll   = 0.060;

Mact_smc = ...
    -sign_Broll*( ...
        K_Mact_lin*s_roll ...
        + K_Mact_sw*satfun(s_roll/phi_roll) );

Mact_smc = clamp(Mact_smc,-Mact_max,Mact_max);

% Blend analytical-model inversion with robust SMC
alpha_roll_model = 0.35;

if abs(B_roll) <= 1.0e-8
    alpha_roll_model = 0.0;
end

Mact_target = ...
      alpha_roll_model*Mact_model ...
    + (1.0-alpha_roll_model)*Mact_smc;

% LTR correction
LTR_on = 0.20;

if abs(LTR_t_model) > LTR_on && abs(B_LTR) > 1.0e-8

    dM_LTR = ...
        -0.20*LTR_t_model/B_LTR;

    dM_LTR = ...
        clamp(dM_LTR,-3000.0,3000.0);

    Mact_target = ...
        Mact_target+dM_LTR;

end

Mact_target = clamp(Mact_target,-Mact_max,Mact_max);

% Straight-road dead zone
if ...
       abs(phi_t)  < 0.0005 ...
    && abs(dphi_t) < 0.0020 ...
    && abs(phi_s)  < 0.0007 ...
    && abs(dphi_s) < 0.0030 ...
    && abs(LTR_t_model) < 0.02

    Mact_target = 0.0;

end

% Smooth actuator
Mact_rate_max = 25000.0;
Mact_step_max = Mact_rate_max*Ts;

Mact_cmd = ...
    rate_limit( ...
        Mact_target, ...
        u_prev(3), ...
        Mact_step_max );

Mact_cmd = clamp(Mact_cmd,-Mact_max,Mact_max);


%% ========================================================================
% 4. SIX-WHEEL SPEED REFERENCES
% ========================================================================

%% Tractor desired lateral velocity
%
% psi_ref is tangent to desired path, so sideslip reference is
% approximately zero. Keep vy_ref = 0 for first baseline.

vy_ref = ...
    0.0;


%% ------------------------------------------------------------------------
% Front axle wheel-plane speeds
% -------------------------------------------------------------------------

VfL_x = ...
    vx_ref ...
    - rt_ref*Tf/2.0;


VfR_x = ...
    vx_ref ...
    + rt_ref*Tf/2.0;


Vf_y = ...
    vy_ref ...
    + rt_ref*Lf;


VfL = ...
      VfL_x*cos(delta_cmd) ...
    + Vf_y*sin(delta_cmd);


VfR = ...
      VfR_x*cos(delta_cmd) ...
    + Vf_y*sin(delta_cmd);


%% ------------------------------------------------------------------------
% Tractor rear axle
% -------------------------------------------------------------------------

VrL = ...
    vx_ref ...
    - rt_ref*Tr/2.0;


VrR = ...
    vx_ref ...
    + rt_ref*Tr/2.0;


%% ------------------------------------------------------------------------
% Trailer
%
% Approximate desired trailer yaw rate:
% rs_ref ~= rt_ref
% -------------------------------------------------------------------------

rs_ref = ...
    rt_ref;


%% Desired articulation approximation

Lrs = ...
    8.500;


vx_ref_safe = ...
    max(abs(vx_ref),3.0);


gamma_ref = ...
    -Lrs*rt_ref/vx_ref_safe;


%% Trailer longitudinal speed approximation

Vxs_ref = ...
    vx_ref*cos(gamma_ref);


VsL = ...
    Vxs_ref ...
    - rs_ref*Ts_track/2.0;


VsR = ...
    Vxs_ref ...
    + rs_ref*Ts_track/2.0;


%% Prevent negative wheel reference

VfL = max(VfL,0.0);
VfR = max(VfR,0.0);

VrL = max(VrL,0.0);
VrR = max(VrR,0.0);

VsL = max(VsL,0.0);
VsR = max(VsR,0.0);


%% Angular-speed references

omega_ref(1) = ...
    VfL/Rf;


omega_ref(2) = ...
    VfR/Rf;


omega_ref(3) = ...
    VrL/Rr;


omega_ref(4) = ...
    VrR/Rr;


omega_ref(5) = ...
    VsL/Rs;


omega_ref(6) = ...
    VsR/Rs;


%% ========================================================================
% WHEEL-SPEED ERRORS
% ========================================================================

ew1 = ...
    omega_fL-omega_ref(1);

ew2 = ...
    omega_fR-omega_ref(2);

ew3 = ...
    omega_rL-omega_ref(3);

ew4 = ...
    omega_rR-omega_ref(4);

ew5 = ...
    omega_sL-omega_ref(5);

ew6 = ...
    omega_sR-omega_ref(6);


%% ========================================================================
% BASE LONGITUDINAL ALLOCATION
% ========================================================================

Tdrive_target = ...
    0.0;


Tb_fL_target = 0.0;
Tb_fR_target = 0.0;

Tb_rL_target = 0.0;
Tb_rR_target = 0.0;

Tb_sL_target = 0.0;
Tb_sR_target = 0.0;


if Fx_target >= 0.0

    %% Propulsion

    Tdrive_target = ...
        Fx_target*Rf;

else

    %% Base braking

    Fb = ...
        -Fx_target;


    wf = 0.35;

    wr = 0.40;

    ws = 0.25;


    Tb_fL_target = ...
        0.5*wf*Fb*Rf;

    Tb_fR_target = ...
        0.5*wf*Fb*Rf;


    Tb_rL_target = ...
        0.5*wr*Fb*Rr;

    Tb_rR_target = ...
        0.5*wr*Fb*Rr;


    Tb_sL_target = ...
        0.5*ws*Fb*Rs;

    Tb_sR_target = ...
        0.5*ws*Fb*Rs;

end


%% ========================================================================
% 4. INDIVIDUAL WHEEL-SPEED SMC
%
% We only have one common drive torque.
%
% Therefore individual wheel control is achieved with differential
% braking.
%
% If wheel is faster than its reference -> add brake torque.
%
% If wheel is slower -> do NOT brake it. Common Tdrive accelerates vehicle.
% ========================================================================

Komega = ...
    350.0;


phi_omega = ...
    1.50;


omega_dead = ...
    0.30;


Tb_fL_target = ...
    Tb_fL_target ...
    + wheel_brake_smc( ...
        ew1, ...
        Komega, ...
        phi_omega, ...
        omega_dead );


Tb_fR_target = ...
    Tb_fR_target ...
    + wheel_brake_smc( ...
        ew2, ...
        Komega, ...
        phi_omega, ...
        omega_dead );


Tb_rL_target = ...
    Tb_rL_target ...
    + wheel_brake_smc( ...
        ew3, ...
        Komega, ...
        phi_omega, ...
        omega_dead );


Tb_rR_target = ...
    Tb_rR_target ...
    + wheel_brake_smc( ...
        ew4, ...
        Komega, ...
        phi_omega, ...
        omega_dead );


Tb_sL_target = ...
    Tb_sL_target ...
    + wheel_brake_smc( ...
        ew5, ...
        Komega, ...
        phi_omega, ...
        omega_dead );


Tb_sR_target = ...
    Tb_sR_target ...
    + wheel_brake_smc( ...
        ew6, ...
        Komega, ...
        phi_omega, ...
        omega_dead );


%% ========================================================================
% PHYSICAL SATURATIONS
% ========================================================================

Tdrive_target = ...
    clamp(Tdrive_target,0.0,8000.0);


Tb_fL_target = ...
    clamp(Tb_fL_target,0.0,6000.0);

Tb_fR_target = ...
    clamp(Tb_fR_target,0.0,6000.0);


Tb_rL_target = ...
    clamp(Tb_rL_target,0.0,6000.0);

Tb_rR_target = ...
    clamp(Tb_rR_target,0.0,6000.0);


Tb_sL_target = ...
    clamp(Tb_sL_target,0.0,6000.0);

Tb_sR_target = ...
    clamp(Tb_sR_target,0.0,6000.0);


%% ========================================================================
% ACTUATOR RATE LIMITS
% ========================================================================

Tdrive_step = ...
    20000.0*Ts;


Tb_step = ...
    30000.0*Ts;


Tdrive_cmd = ...
    rate_limit( ...
        Tdrive_target, ...
        u_prev(2), ...
        Tdrive_step );


Tb_fL = ...
    rate_limit( ...
        Tb_fL_target, ...
        u_prev(4), ...
        Tb_step );


Tb_fR = ...
    rate_limit( ...
        Tb_fR_target, ...
        u_prev(5), ...
        Tb_step );


Tb_rL = ...
    rate_limit( ...
        Tb_rL_target, ...
        u_prev(6), ...
        Tb_step );


Tb_rR = ...
    rate_limit( ...
        Tb_rR_target, ...
        u_prev(7), ...
        Tb_step );


Tb_sL = ...
    rate_limit( ...
        Tb_sL_target, ...
        u_prev(8), ...
        Tb_step );


Tb_sR = ...
    rate_limit( ...
        Tb_sR_target, ...
        u_prev(9), ...
        Tb_step );


%% ========================================================================
% OUTPUT
% ========================================================================

u9(1) = ...
    delta_cmd;


u9(2) = ...
    Tdrive_cmd;


%% Active roll moment

u9(3) = ...
    Mact_cmd;


u9(4) = ...
    Tb_fL;


u9(5) = ...
    Tb_fR;


u9(6) = ...
    Tb_rL;


u9(7) = ...
    Tb_rR;


u9(8) = ...
    Tb_sL;


u9(9) = ...
    Tb_sR;


end


%% =========================================================================
% REFERENCE GENERATOR
% =========================================================================

function [vx_ref,ax_ref,Y_ref,dY_ref,psi_ref,rt_ref] = ...
    reference_local(t)
%#codegen


%% ========================================================================
% SPEED REFERENCE FOR ACCELERATION + BRAKING TEST
% ========================================================================

v0 = 40.0/3.6;     % 11.11 m/s

if t < 5.0

    % Accelerate
    ax_ref = 0.40;

    vx_ref = ...
        v0 + ax_ref*t;

elseif t < 10.0

    % Hold speed
    ax_ref = 0.0;

    vx_ref = ...
        v0 + 0.40*5.0;

elseif t < 16.0

    % BRAKING TEST
    ax_ref = -0.60;

    vx_ref = ...
        v0 ...
        + 0.40*5.0 ...
        - 0.60*(t-10.0);

else

    % Hold after braking
    ax_ref = 0.0;

    vx_ref = ...
        v0 ...
        + 0.40*5.0 ...
        - 0.60*6.0;

end


%% Double lane change

A = 1.75;

t1 = 6.5;

t2 = 14.75;

w = 1.0;


z1 = ...
    (t-t1)/w;


z2 = ...
    (t-t2)/w;


th1 = ...
    tanh(z1);


th2 = ...
    tanh(z2);


Y_ref = ...
    A*(th1-th2);


q1 = ...
    1.0-th1*th1;


q2 = ...
    1.0-th2*th2;


dY_ref = ...
    (A/w)*(q1-q2);


ddY_ref = ...
    (A/(w*w))*( ...
       -2.0*th1*q1 ...
       +2.0*th2*q2 );


vx_safe = ...
    max(abs(vx_ref),1.0);


psi_ref = ...
    atan2( ...
        dY_ref, ...
        vx_safe );


num = ...
      vx_safe*ddY_ref ...
    - dY_ref*ax_ref;


den = ...
      vx_safe*vx_safe ...
    + dY_ref*dY_ref;


rt_ref = ...
    num/max(den,1.0e-6);


end


%% =========================================================================
% WHEEL BRAKE SMC
% =========================================================================

function Tb = wheel_brake_smc( ...
    ew, ...
    Komega, ...
    phi_omega, ...
    deadband)
%#codegen


if ew <= deadband

    Tb = ...
        0.0;

else

    s = ...
        (ew-deadband)/phi_omega;


    Tb = ...
        Komega*satfun(s);

end


end


%% =========================================================================
% SATURATION FUNCTION
% =========================================================================

function y = satfun(z)
%#codegen


if z > 1.0

    y = 1.0;

elseif z < -1.0

    y = -1.0;

else

    y = z;

end


end


%% =========================================================================
% RATE LIMITER
% =========================================================================

function y = rate_limit( ...
    target, ...
    previous, ...
    max_step)
%#codegen


d = ...
    target-previous;


if d > max_step

    d = max_step;

elseif d < -max_step

    d = -max_step;

end


y = ...
    previous+d;


end


%% =========================================================================
% CLAMP
% =========================================================================

function y = clamp(x,xmin,xmax)
%#codegen


if x > xmax

    y = xmax;

elseif x < xmin

    y = xmin;

else

    y = x;

end


end


%% =========================================================================
% ANGLE WRAP
% =========================================================================

function a = wrap_pi(a)
%#codegen


a = ...
    atan2( ...
        sin(a), ...
        cos(a) );


end

== matlab function roll_model_TRUCKSIM_18DOF_REVISED/Subsystem2/MATLAB Function4 ==
  data: ref12 input; dX_ref output; dY_ref output
function [dX_ref,dY_ref] = fcn(ref12)
%#codegen

v   = ref12(1);
psi = ref12(5);

dX_ref = v*cos(psi);
dY_ref = v*sin(psi);
end

== matlab function roll_model_TRUCKSIM_18DOF_REVISED/TRUCKSIM MODEL VALIDATION/Subsystem2/Subsystem/MATLAB Function1 ==
  data: v input; dX_ref output; dY_ref output; psi input
function [dX_ref,dY_ref] = fcn(v,psi)
%#codegen


dX_ref = v*cos(psi);
dY_ref = v*sin(psi);
end

== matlab function roll_model_TRUCKSIM_18DOF_REVISED/Subsystem2/MATLAB Function5 ==
  data: Fy6_raw input; Fy6_alloc output; Fy6_view output
function [Fy6_alloc,Fy6_view] = fcn(Fy6_raw)
%#codegen

persistent FyFilt

if isempty(FyFilt)
    FyFilt = zeros(6,1);
end

Ts  = 0.01;
tau = 0.15;

alpha = Ts/(tau+Ts);

FyFilt = FyFilt + alpha*(Fy6_raw-FyFilt);

Fy6_alloc = Fy6_raw;
Fy6_view  = FyFilt;

end

== matlab function roll_model_TRUCKSIM_18DOF_REVISED/TRUCKSIM MODEL VALIDATION/Subsystem2/MATLAB Function ==
  data: rt input; gamma_dot output; rs input; psi_dot output
function [gamma_dot,psi_dot] = fcn(rt,rs)
gamma_dot = rt - rs;
psi_dot = rt;

== matlab function roll_model_TRUCKSIM_18DOF_REVISED/TRUCKSIM MODEL VALIDATION/Subsystem2/MATLAB Function1 ==
  data: u input; y output; t input
function y = fcn(u,t)

if t < 2e-3
    y = u + 0.1;
else
    y = u;
end

== matlab function roll_model_TRUCKSIM_18DOF_REVISED/TRUCKSIM MODEL VALIDATION/Subsystem2/MATLAB Function2 ==
  data: vxt input; y output; vyt input
function y = fcn(vxt,vyt)

y = vxt/vyt;

== matlab function roll_model_TRUCKSIM_18DOF_REVISED/TRUCKSIM MODEL VALIDATION/Subsystem2/Subsystem/MATLAB Function ==
  data: rt input; gamma_dot output; rs input; psi_dot output
function [gamma_dot,psi_dot] = fcn(rt,rs)
gamma_dot = rt - rs;
psi_dot = rt;
